simulink model "supervisor"  (R2026a)
settings: configuration reference "MCConfiguration" (kept outside this file)
settings Model: DataDictionary=embeddedBoard_common.sldd  SimulationMode=accelerator  Creator=mfussi  LastModifiedBy=rpumpo
settings ConfigSetRef: SourceName=MCConfiguration

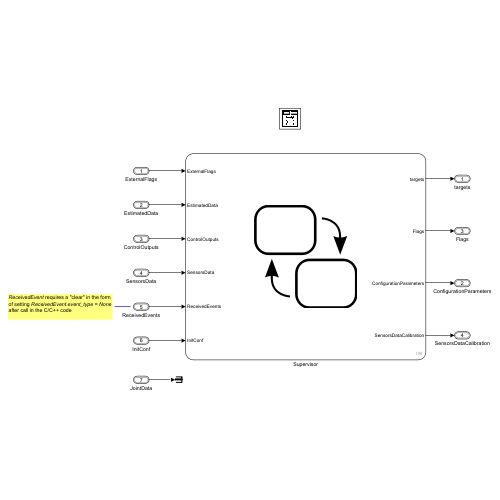
[thumbnail: Simulink's stored preview of the top-level diagram]
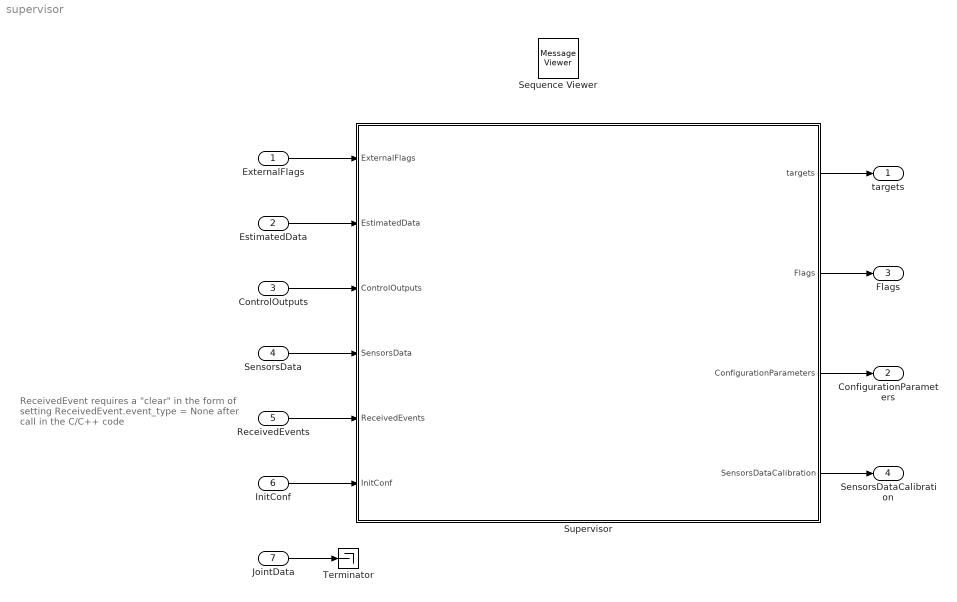
== system supervisor ==
  note: ReceivedEvent requires a "clear" in the form of setting ReceivedEvent.event_type = None after call in the C/C++ code
  ExternalFlags : Inport  OutDataTypeStr=Bus: ExternalFlags  BusOutputAsStruct=on
  EstimatedData : Inport  Port=2  OutDataTypeStr=Bus: EstimatedData  BusOutputAsStruct=on
  ControlOutputs : Inport  Port=3  OutDataTypeStr=Bus: FOCOutputs  BusOutputAsStruct=on
  SensorsData : Inport  Port=4  OutDataTypeStr=Bus: SensorsData  BusOutputAsStruct=on
  ReceivedEvents : Inport  Description=|  Port=5  OutDataTypeStr=Bus: ReceivedEvents  BusOutputAsStruct=on
      | ReceivedEvent requires a "clear" 
      | in the form of setting ReceivedEvent.event_type = None after call in the C/C++ code
  InitConf : Inport  Port=6  OutDataTypeStr=Bus: ActuatorConfiguration  BusOutputAsStruct=on
  JointData : Inport  Port=7  OutDataTypeStr=Bus: JointData
  Sequence Viewer : MessageViewer  History=1000  SavedRootId=#
  Supervisor : Stateflow chart  TreatAsAtomicUnit=on
      settings: PortSchema="{\"entries\":[{\"content\":{\"sides\":[{\"content\":{\"connectorIds\":[\"In2\",\"In1\",\"In3\",\"In4\",\"In6\",\"In5\"]},\"type\":\"ConnectorPlacement.EquallySpacedRectSide\",\"uuid\":\"924267b7-0662-4a36-add4-8ce875a6673d\"},{\"content\":{\"connectorIds\":[\"Out1\",\"Out2\",\"Out3\",\"Out4\"],\"side\":\"RIGHT\"},\"type\":\"ConnectorPlacement.EquallySpacedRectSide\",\"uuid\":\"edfdb85b-b8c0-45b0-9100-5f30a86fff38\"},{\"content\":{\"side\":\"TOP\"},\"type\":\"ConnectorPlacement.EquallySpacedRectSide\",\"uuid\":\"ff8cc695-ae52-41b0-91e9-1dc41b5aad3d\"},{\"content\":{\"side\":\"BOTTOM\"},\"type\":\"ConnectorPlacement.EquallySpacedRectSide\",\"uuid\":\"f5fe8171-8dce-40c2-ade3-2941f2e0d5a7\"}]},\"type\":\"ConnectorPlacement.EquallySpacedConnector\",\"uuid\":\"ae0a1b0b-beda-484a-966c-3dd739fb9179\"}],\"packageUris\":[\"http://schema.mathworks.com/mf0/Connector/R2020b\"],\"version\":\"1.0\"}"
  Terminator : Terminator
  targets : Outport  OutDataTypeStr=Bus: Targets  BusOutputAsStruct=on
  ConfigurationParameters : Outport  Port=2  OutDataTypeStr=Bus: ActuatorConfiguration  BusOutputAsStruct=on
  Flags : Outport  Port=3  OutDataTypeStr=Bus: Flags  BusOutputAsStruct=on
  SensorsDataCalibration : Outport  Port=4  OutDataTypeStr=Bus: SensorsData  BusOutputAsStruct=on
  wires:
  ExternalFlags/1 -> Supervisor/2(ExternalFlags)
  EstimatedData/1 -> Supervisor/1(EstimatedData)
  ControlOutputs/1 -> Supervisor/3(ControlOutputs)
  SensorsData/1 -> Supervisor/4(SensorsData)
  ReceivedEvents/1 -> Supervisor/6(ReceivedEvents)
  Supervisor/1(targets) -> targets/1
  Supervisor/3(ConfigurationParameters) -> ConfigurationParameters/1
  Supervisor/2(Flags) -> Flags/1
  InitConf/1 -> Supervisor/5(InitConf)
  JointData/1 -> Terminator/1
  Supervisor/4(SensorsDataCalibration) -> SensorsDataCalibration/1

== stateflow chart supervisor/Supervisor ==
  settings: updateMethod=DISCRETE  sampleTime=Ts_Supervision
  state FaultsManager [parallel]
    settings: executionOrder=1
    state FaultButton [parallel]
      settings: executionOrder=2
      state NoFault
        entry:
        isFaultButtonPressed = false;
      state ButtonPressed
        entry:
        isFaultButtonPressed = true;
      (default) -> FaultsManager.FaultButton.NoFault
      ButtonPressed -> FaultsManager.FaultButton.NoFault : [hasChangedTo(ExternalFlags.fault_button, false)]
      FaultsManager.FaultButton.NoFault -> ButtonPressed : [hasChangedTo(ExternalFlags.fault_button, true)]
    state HWFaults [parallel]
      settings: executionOrder=1
      state NoFault
        entry:
        isInFault=false;
        Flags.hw_faults.overcurrent = false;
      state LimitNonConfigured
      state OverCurrentFault
        entry:
        Flags.hw_faults.overcurrent = true;
        isInFault=true;
      (default) -> LimitNonConfigured
      LimitNonConfigured -> FaultsManager.HWFaults.NoFault : [areLimitsSet==true]
      FaultsManager.HWFaults.NoFault -> OverCurrentFault : [abs(EstimatedData.Iq_filtered) >= ConfigurationParameters.thresholds.motorOverloadCurrents]
      OverCurrentFault -> FaultsManager.HWFaults.NoFault : [abs(EstimatedData.Iq_filtered) < ConfigurationParameters.thresholds.motorOverloadCurrents]
  state ControlModeHandler [parallel]
    settings: executionOrder=2
    state Calibration
      entry:
      Flags.control_mode = ControlModes.Current;
      during :
      SensorsDataCalibration.motorsensors.Iabc = SensorsData.motorsensors.Iabc;
      state p_idx_out =CheckIdx(idx,p_idx) [function]
        (default) -> (junction 1789) : {diff_index = idx - p_idx;}
        (junction 1789) -> (junction 1791) [order 1] : [diff_index ~= 0]{p_idx_out = idx;}
        (junction 1789) -> (junction 1791) [order 2]
      state computed_offset = ComputeOffset(angle) [function]
        (default) -> (junction 1799) : {computed_offset = 45 - angle;}
        (junction 1799) -> (junction 1800) [order 1] : [computed_offset >360]{computed_offset = computed_offset -360;}
        (junction 1799) -> (junction 1800) [order 2]
      state Zero_electric
        entry:
        finish = false;
        p_index = SensorsData.motorsensors.qencoder.Idx_counter;
        diff_index = 0;
        tzeroalign = 0.7;
        talign = 0.01;
        v_threshold = 1;
        count = 0;
        SensorsDataCalibration.motorsensors.electrical_angle = count;
      state Search_idx
        entry:
        count = count+1;
        SensorsDataCalibration.motorsensors.electrical_angle = count;
        p_index = CheckIdx(SensorsData.motorsensors.qencoder.Idx_counter,p_index);
      state velocity_check
        newSetpoint = ConfigurationParameters.thresholds.motorNominalCurrents;
        send(ControlModeSetpointChange, TargetsManager);
      state Idx_found
        entry:
        SensorsDataCalibration.motorsensors.electrical_angle = 0;
      state Finish
        newSetpoint = 0;
        send(ControlModeSetpointChange, TargetsManager);
      state Read_0_encoder
        entry:
        offset = ComputeOffset(SensorsData.motorsensors.qencoder.rotor_angle);
      (default) -> Zero_electric : {SensorsDataCalibration = SensorsData;}
      Zero_electric -> velocity_check : [Flags.calibration_type ~= CalibrationTypes.None]{condition=1;}
      Search_idx -> Zero_electric [order 1] : [count == 360]
      velocity_check -> Search_idx [order 3] : [after(tzeroalign,sec)&& condition ==1]
      Search_idx -> velocity_check [order 3] : {condition=2;}
      velocity_check -> Search_idx [order 4] : [after(talign,sec)&&condition ==2]
      velocity_check -> velocity_check [order 2] : [abs(EstimatedData.rotor_velocity) >v_threshold]
      Search_idx -> Finish [order 2] : [diff_index~=0 && Flags.calibration_type== CalibrationTypes.Search_Index]
      velocity_check -> velocity_check [order 1] : [diff_index~=0 && Flags.calibration_type== CalibrationTypes.Full_Calibration && condition ==2]{condition= 3;}
      velocity_check -> Idx_found [order 5] : [after(talign,sec) && condition ==3]
      Idx_found -> velocity_check : {condition = 4;}
      Finish -> (junction 1818) : [after(0.1,sec)]{finish = true;}
      Read_0_encoder -> Finish
      velocity_check -> Read_0_encoder [order 6] : [after(tzeroalign,sec) && condition ==4]
    state NotConfigured
      entry:
      Flags.control_mode = ControlModes.NotConfigured;
      Flags.emit_offset_calibration = false;
      rtw_disableMotor();
    state Idle
      entry:
      Flags.control_mode = ControlModes.Idle;
      rtw_disableMotor();
      //this updates the targets value
      send(ControlModeSetpointChange, TargetsManager);
    state Position
      entry:
      Flags.control_mode = ControlModes.Position;
      newSetpoint = SensorsData.motorsensors.qencoder.rotor_angle;
      trajectoryVelocity = single(1);
      send(ControlModeSetpointChange, TargetsManager);
    state Current
      entry:
      Flags.control_mode = ControlModes.Current;
      send(ControlModeSetpointChange, TargetsManager);
    state HWFault
      entry:
      Flags.control_mode = ControlModes.HwFaultCM;
      rtw_disableMotor();
      //this updates the targets value
      send(ControlModeSetpointChange, TargetsManager);
    note: IMPORTANT:
        | Currently we use IDLE command to exit from HWFault state,
        | but We should use FORCE_IDLE command when it will be implemented
    state Voltage
      entry:
      Flags.control_mode = ControlModes.Voltage;
      send(ControlModeSetpointChange, TargetsManager);
    state Velocity
      entry:
      Flags.control_mode = ControlModes.Velocity;
      send(ControlModeSetpointChange, TargetsManager);
    (default) -> NotConfigured : {ConfigurationParameters = InitConf;}
    Calibration -> (junction 233) [order 2] : [finish]{Flags.calibration_type = CalibrationTypes.None; Flags.calibration_done = true;}
    Idle -> Calibration [order 1] : EnableCalibration
    Calibration -> (junction 233) [order 1] : [finish && Flags.calibration_type == CalibrationTypes.Full_Calibration]{Flags.calibration_type = CalibrationTypes.None; Flags.calibration_done = true;
        | ConfigurationParameters.motor.externals.rotor_index_offset = offset;
        |  Flags.emit_offset_calibration = true;}
    NotConfigured -> (junction 229) [order 1] : initialControlModeTrigger
        | {requestedControlMode = ControlModes.Idle;}
    (junction 229) -> (junction 233)
    (junction 227) -> (junction 233)
    (junction 273) -> (junction 229)
    (junction 233) -> Idle
    (junction 282) -> (junction 227)
    HWFault -> NotConfigured [order 1] : [!isInFault &&  ...
        | isReqMode(ControlModes.Idle) && ...
        | !isConfigurationSet()]
    NotConfigured -> HWFault [order 2] : [isInFault]
    (junction 228) -> Idle
    (junction 236) -> (junction 228)
    Idle -> (junction 230) [order 3] : [!isReqMode(ControlModes.Idle)]
        | {rtw_enableMotor();}
    (junction 230) -> (junction 237)
    (junction 234) -> Idle : SetCtrlMode[isReqMode(ControlModes.Idle)]
    (junction 235) -> (junction 234) [order 2]
    (junction 224) -> Idle : SetCtrlMode[isReqMode(ControlModes.Idle)]
    (junction 243) -> (junction 224) [order 2]
    (junction 231) -> Idle : SetCtrlMode[isReqMode(ControlModes.Idle)]
    (junction 241) -> (junction 231) [order 2]
    Idle -> (junction 232) [order 2] : [isInFault || isFaultButtonPressed]
    (junction 232) -> (junction 225)
    (junction 225) -> (junction 248)
    Position -> (junction 236) [order 3] : SetCtrlMode[isReqMode(ControlModes.Idle)]
    (junction 237) -> Position [order 1] : SetCtrlMode[isReqMode(ControlModes.Position)]
    (junction 237) -> (junction 244) [order 2]
    (junction 235) -> Position [order 1] : SetCtrlMode[isReqMode(ControlModes.Position)]
    (junction 245) -> (junction 235)
    Position -> (junction 242) [order 2] : SetCtrlMode[!isReqMode(ControlModes.Idle)]
    (junction 242) -> (junction 240)
    (junction 243) -> Position [order 1] : SetCtrlMode[isReqMode(ControlModes.Position)]
    (junction 247) -> (junction 243) [order 2]
    (junction 241) -> Position [order 1] : SetCtrlMode[isReqMode(ControlModes.Position)]
    (junction 255) -> (junction 241) [order 2]
    Position -> (junction 238) [order 1] : [isInFault || isFaultButtonPressed]
    (junction 238) -> (junction 248)
    (junction 248) -> (junction 259)
    (junction 244) -> Current [order 1] : SetCtrlMode[isReqMode(ControlModes.Current)]{ newSetpoint=0; }
    (junction 244) -> (junction 278) [order 2]
    Current -> (junction 245) [order 3]
    (junction 240) -> (junction 239) [order 1] : SetCtrlMode[isReqMode(ControlModes.Current)]
    (junction 239) -> Current : {newSetpoint=EstimatedData.Iq_filtered;}
    (junction 240) -> (junction 258) [order 2]
    (junction 247) -> (junction 246) [order 1] : SetCtrlMode[isReqMode(ControlModes.Current)]
    (junction 246) -> (junction 276)
    (junction 263) -> (junction 247)
    Current -> (junction 275) [order 2] : SetCtrlMode[!isReqMode(ControlModes.Idle) && !isReqMode(ControlModes.Position)]
    (junction 275) -> (junction 257)
    (junction 276) -> Current : {newSetpoint=EstimatedData.Iq_filtered;}
    (junction 255) -> (junction 276) [order 1] : SetCtrlMode[isReqMode(ControlModes.Current)]
    (junction 261) -> (junction 255) [order 2]
    HWFault -> (junction 273) [order 2] : SetCtrlMode[!isInFault && isReqMode(ControlModes.Idle)]
    Current -> (junction 267) [order 1] : [isInFault || isFaultButtonPressed]
    (junction 268) -> HWFault
    (junction 267) -> (junction 259)
    (junction 259) -> (junction 279)
    (junction 278) -> Voltage [order 1] : SetCtrlMode[isReqMode(ControlModes.Voltage)]
        | {newSetpoint=0; }
    (junction 278) -> (junction 251) [order 2]
    (junction 258) -> (junction 277) [order 1] : SetCtrlMode[isReqMode(ControlModes.Voltage)]
    (junction 277) -> Voltage : {newSetpoint=ControlOutputs.Vq;}
    (junction 258) -> (junction 251) [order 2]
    (junction 283) -> (junction 277)
    Voltage -> (junction 263) [order 2]
    (junction 257) -> (junction 283) [order 1] : SetCtrlMode[isReqMode(ControlModes.Voltage)]
    (junction 257) -> (junction 251) [order 2]
    Voltage -> (junction 251) [order 3]
    (junction 269) -> Voltage : {newSetpoint=ControlOutputs.Vq;}
    (junction 261) -> (junction 269) [order 1] : SetCtrlMode[isReqMode(ControlModes.Voltage)]
    (junction 265) -> (junction 261) : SetCtrlMode[!isReqMode(ControlModes.Velocity)]
    Voltage -> (junction 260) [order 1] : [isInFault || isFaultButtonPressed]
    (junction 260) -> (junction 279)
    (junction 279) -> (junction 253)
    (junction 251) -> Velocity : SetCtrlMode[isReqMode(ControlModes.Velocity)]
        | {newSetpoint=EstimatedData.rotor_velocity;}
    Velocity -> (junction 265) [order 2]
    Velocity -> (junction 280) [order 1] : [isInFault || isFaultButtonPressed]
    (junction 280) -> (junction 253)
    (junction 253) -> (junction 281)
    (junction 281) -> (junction 268) [order 1] : [isInFault]
    (junction 281) -> (junction 282) [order 2] : [isFaultButtonPressed]
  state TargetsManager [parallel]
    settings: executionOrder=4
    state ResetTargets [function]
      (default) -> (junction 1055) : {targets.voltage = 0;
          | targets.current = 0;
          | targets.velocity = 0;
          | targets.position = 0;
          | targets.trajectory_time = 0; }
    state Home
    (default) -> TargetsManager.Home : {ResetTargets();}
    (junction 968) -> TargetsManager.Home [order 1] : [in(ControlModeHandler.Current)| in(ControlModeHandler.Calibration)]
        | {targets.current = newSetpoint;}
    (junction 968) -> TargetsManager.Home [order 5] : [in(ControlModeHandler.Position)]
        | {targets.position = newSetpoint;
        | targets.velocity = trajectoryVelocity;}
    (junction 968) -> TargetsManager.Home [order 2] : [in(ControlModeHandler.Voltage)]
        | {targets.voltage = newSetpoint;}
    (junction 968) -> TargetsManager.Home [order 4] : [in(ControlModeHandler.Velocity)]
        | {targets.velocity = newSetpoint;}
    TargetsManager.Home -> (junction 968) [order 2] : DispatcherSetpointChange
    TargetsManager.Home -> (junction 968) [order 1] : ControlModeSetpointChange
    (junction 968) -> TargetsManager.Home [order 3] : [in(ControlModeHandler.Idle) || ...
        | in(ControlModeHandler.HWFault)]
        | {ResetTargets();}
    (junction 968) -> TargetsManager.Home [order 6] : //Default Transition
  state ConfigurationManager [parallel]
    settings: executionOrder=5
    state Home
      entry:
      param_is_set = false;
      cfg_is_set = false;
    state SetExternalConfig
      entry:
      cfg_is_set = true;
    state SetConfigParam
      entry:
      param_is_set = true;
    state wait_required = SetMotorParam(cfg_set) [function]
      (default) -> (junction 1841)
      (junction 1841) -> (junction 1842) [order 1] : [cfg_set.key == MCMotorParamsSet.Kbemf]
      (junction 1841) -> (junction 1845) [order 2]
      (junction 1842) -> (junction 1843) : {ConfigurationParameters.motor.Kbemf = cfg_set.value[0][0];
          | wait_required  = false;}
      (junction 1843) -> (junction 1844)
      (junction 1844) -> (junction 1848)
      (junction 1845) -> (junction 1846) [order 1] : [cfg_set.key == MCMotorParamsSet.elect_vmax]
      (junction 1845) -> (junction 1849) [order 2]
      (junction 1846) -> (junction 1847) : {ConfigurationParameters.motor.Vmax = cfg_set.value[0][0];
          | wait_required  = false;}
      (junction 1847) -> (junction 1848)
      (junction 1848) -> (junction 1853)
      (junction 1849) -> (junction 1850) [order 1] : [cfg_set.key == MCMotorParamsSet.hall]
      (junction 1849) -> (junction 1854) [order 2]
      (junction 1850) -> (junction 1852) : {ConfigurationParameters.motor.hall_sensors_offset = cfg_set.value[0][0];
          | ConfigurationParameters.motor.hall_sensors_swapBC = cfg_set.value[1][0];
          | wait_required  = true;}
      (junction 1852) -> (junction 1853)
      (junction 1854) -> (junction 1851)
      (junction 1853) -> (junction 1855)
      (junction 1855) -> (junction 1854)
    state CheckCalibration(motor_config) [function]
      (junction 1879) -> (junction 1878) : {offset = motor_config.rotor_index_offset;
          | has_index = motor_config.has_quadrature_encoder;}
      (default) -> (junction 1879)
      (junction 1878) -> (junction 1880)
      (junction 1880) -> (junction 1883) [order 2] : {Flags.calibration_done = true;}
      (junction 1880) -> (junction 1881) [order 1] : [has_index]{Flags.calibration_done = false;}
      (junction 1881) -> (junction 1882) [order 1] : [offset == -1]
          | {Flags.calibration_type= CalibrationTypes.Full_Calibration;}
      (junction 1881) -> (junction 1882) [order 2] : {Flags.calibration_type = CalibrationTypes.Search_Index;}
      (junction 1882) -> (junction 1883) : {send(EnableCalibration,ControlModeHandler);}
    (default) -> ConfigurationManager.Home
    ConfigurationManager.Home -> ConfigurationManager.Home [order 3] : SetMotorParam
        | [!SetMotorParam(temp_config_set)]
    ConfigurationManager.Home -> SetExternalConfig [order 1] : SetMotorConfigExternal
        | {ConfigurationParameters.motor.externals = temp_motor_config;}
    SetExternalConfig -> ConfigurationManager.Home [order 5] : [cfg_is_set]
        | {hardwareConfigMotor(motor_id_to_configure);
        | CheckCalibration(temp_motor_config);}
    SetExternalConfig -> ConfigurationManager.Home [order 1] : [hasChanged(motor_id_to_configure)]
    ConfigurationManager.Home -> SetConfigParam [order 2] : SetMotorParam
        | [SetMotorParam(temp_config_set)]
    SetConfigParam -> ConfigurationManager.Home [order 3] : [cfg_is_set]
        | {hardwareConfigMotor(motor_id_to_configure);
        | CheckCalibration(temp_motor_config);}
    SetConfigParam -> ConfigurationManager.Home [order 1] : [hasChanged(motor_id_to_configure)]
    SetExternalConfig -> SetExternalConfig [order 3] : SetMotorConfigExternal
        | {ConfigurationParameters.motor.externals = temp_motor_config;}
    SetExternalConfig -> SetExternalConfig [order 4] : SetMotorParam[!SetMotorParam(temp_config_set)]
    SetConfigParam -> SetExternalConfig [order 2] : SetMotorConfigExternal
        | {ConfigurationParameters.motor.externals = temp_motor_config;}
    SetExternalConfig -> SetConfigParam [order 2] : SetMotorParam[SetMotorParam(temp_config_set)]
    SetConfigParam -> SetConfigParam [order 4] : SetMotorParam
        | {SetMotorParam(temp_config_set);}
  state InputsDispatcher [parallel]
    settings: executionOrder=3
    state SetPid(pid) [function]
      (default) -> (junction 1523)
      (junction 1523) -> (junction 1522) [order 5]
      (junction 1523) -> (junction 1527) [order 4] : [pid.type == ControlModes.Velocity]
      (junction 1523) -> (junction 1526) [order 3] : [pid.type == ControlModes.Voltage]
      (junction 1523) -> (junction 1524) [order 1] : [pid.type == ControlModes.Current]
      (junction 1522) -> (junction 1528)
      (junction 1523) -> (junction 1525) [order 2] : [pid.type == ControlModes.Position]
      (junction 1526) -> (junction 1531) : {DirectPID.P = pid.P;
          | DirectPID.I = pid.I;
          | DirectPID.D = pid.D;
          | DirectPID.shift_factor = pid.shift_factor;}
      (junction 1527) -> (junction 1529) : {ConfigurationParameters.pids.velocityPID.P = pid.P;
          | ConfigurationParameters.pids.velocityPID.I = pid.I;
          | ConfigurationParameters.pids.velocityPID.D = pid.D;
          | ConfigurationParameters.pids.velocityPID.shift_factor = pid.shift_factor;}
      (junction 1524) -> (junction 1530) : {ConfigurationParameters.pids.currentPID.P = pid.P;
          | ConfigurationParameters.pids.currentPID.I = pid.I;
          | ConfigurationParameters.pids.currentPID.D = pid.D;
          | ConfigurationParameters.pids.currentPID.shift_factor = pid.shift_factor;
          | ConfigurationParameters.pids.currentPID.type = ControlModes.Current;}
      (junction 1525) -> (junction 1532) : {ConfigurationParameters.pids.positionPID.P = pid.P;
          | ConfigurationParameters.pids.positionPID.I = pid.I;
          | ConfigurationParameters.pids.positionPID.D = pid.D;
          | ConfigurationParameters.pids.positionPID.shift_factor = pid.shift_factor;
          | ConfigurationParameters.pids.positionPID.type = ControlModes.Position;}
      (junction 1528) -> (junction 1529)
      (junction 1529) -> (junction 1531)
      (junction 1531) -> (junction 1532)
      (junction 1530) -> (junction 1532)
    state SetTarget(tg) [function]
      (junction 1501) -> (junction 1499) [order 1] : [in(ControlModeHandler.Voltage)]{newSetpoint = tg.voltage;}
      (junction 1499) -> (junction 1500)
      (junction 1501) -> (junction 1500) [order 2] : [in(ControlModeHandler.Current)]{newSetpoint = tg.current;}
      (junction 1500) -> (junction 1502)
      (junction 1501) -> (junction 1502) [order 3] : [in(ControlModeHandler.Velocity)]{newSetpoint = tg.velocity;}
      (default) -> (junction 1501)
      (junction 1501) -> (junction 1805) [order 4] : [in(ControlModeHandler.Position)]
          | {newSetpoint = tg.position; trajectoryVelocity = tg.velocity;}
      (junction 1501) -> (junction 1503) [order 5] : [!in(ControlModeHandler.Calibration)]{newSetpoint = 0;}
      (junction 1502) -> (junction 1805)
      (junction 1805) -> (junction 1503)
      (junction 1503) -> (junction 1504) : {send(DispatcherSetpointChange, TargetsManager);}
    state SetLimits(limits) [function]
      (default) -> (junction 1516) : {ConfigurationParameters.thresholds.motorNominalCurrents = abs(limits.nominal);
          | ConfigurationParameters.thresholds.motorPeakCurrents = abs(limits.peak);
          | ConfigurationParameters.thresholds.motorOverloadCurrents = abs(limits.overload);}
      (junction 1516) -> (junction 1517) : [areLimitsSet == false]
          | {areLimitsSet = true;
          | send(initialControlModeTrigger, ControlModeHandler);}
    state Home
    (default) -> (junction 1161) : /* Consume N events per tick */
    InputsDispatcher.Home -> (junction 1161) : {Flags.enable_sending_msg_status = false;}
    (junction 1161) -> (junction 1165) : {ei = 0;}
    (junction 1165) -> (junction 1432) [order 1] : [ei < MAX_EVENTS_PER_TICK]
    (junction 1432) -> (junction 1433) [order 1] : [ReceivedEvents[ei].event_type == EventTypes.SetLimit]
        | {SetLimits(ReceivedEvents[ei].limits_content);}
    (junction 1414) -> (junction 1165) : {ei++;}
    (junction 1165) -> InputsDispatcher.Home [order 2]
    (junction 1432) -> (junction 1434) [order 2]
    (junction 1433) -> (junction 1435)
    (junction 1434) -> (junction 1435) [order 1] : [ReceivedEvents[ei].event_type == EventTypes.SetPid]
        | {SetPid(ReceivedEvents[ei].pid_content);}
    (junction 1434) -> (junction 1436) [order 2]
    (junction 1435) -> (junction 1437)
    (junction 1436) -> (junction 1437) [order 1] : [ReceivedEvents[ei].event_type == EventTypes.SetMotorConfig]
        | {temp_motor_config = ReceivedEvents[ei].motor_config_content;
        | motor_id_to_configure = ReceivedEvents[ei].motor_id;
        | send(SetMotorConfigExternal, ConfigurationManager);}
    (junction 1436) -> (junction 1438) [order 2]
    (junction 1437) -> (junction 1420)
    (junction 1438) -> (junction 1420) [order 1] : [ReceivedEvents[ei].event_type == EventTypes.SetTarget]
        | {Flags.enable_sending_msg_status = true;
        | SetTarget(ReceivedEvents[ei].targets_content);}
    (junction 1438) -> (junction 1439) [order 2]
    (junction 1420) -> (junction 1431)
    (junction 1439) -> (junction 1431) [order 1] : [ReceivedEvents[ei].event_type == EventTypes.SetControlMode]
        | {requestedControlMode = ReceivedEvents[ei].control_mode_content;
        | send(SetCtrlMode, ControlModeHandler);}
    (junction 1439) -> (junction 1904) [order 2]
    (junction 1431) -> (junction 1903)
    (junction 1904) -> (junction 1903) [order 1] : [ReceivedEvents[ei].event_type == EventTypes.SetMotorParam]
        | {temp_config_set = ReceivedEvents[ei].motor_config_set;
        | motor_id_to_configure = ReceivedEvents[ei].motor_id;
        | send(SetMotorParam, ConfigurationManager);}
    (junction 1904) -> (junction 1417) [order 2]
    (junction 1903) -> (junction 1416)
    (junction 1417) -> (junction 1416) [order 1] : [ReceivedEvents[ei].event_type == EventTypes.None]
        | { /*Skip event */ ;}
    (junction 1416) -> (junction 1414)
    (junction 1417) -> (junction 1414) [order 2]
  data: idx function_input single; p_idx function_input single; p_idx_out function_output single; angle function_input single; computed_offset function_output single; isSet function_output boolean; mode function_input Enum: ControlModes; out function_output boolean; cfg_set function_input Bus: MotorConfigurationExtSet size=1; wait_required function_output boolean; motor_id function_input uint8; motor_config function_input Bus: MotorConfigurationExternal; pid function_input Bus: PID; tg function_input Bus: Targets; limits function_input Bus: SupervisorInputLimits; ei local int32 =0; areLimitsSet local boolean; EstimatedData input Bus: EstimatedData; ExternalFlags input Bus: ExternalFlags; ControlOutputs input Bus: FOCOutputs; targets output Bus: Targets; SensorsData input Bus: SensorsData; isFaultButtonPressed local double; isInFault local double; requestedControlMode local Enum: ControlModes; newSetpoint local double; DirectPID local Bus: PID; Flags output Bus: Flags; InitConf input Bus: ActuatorConfiguration; ReceivedEvents input Bus: ReceivedEvents size=MAX_EVENTS_PER_TICK; MAX_EVENTS_PER_TICK parameter size=1; ConfigurationParameters output Bus: ActuatorConfiguration; offset local double; has_index local double; SensorsDataCalibration output Bus: SensorsData; condition local double; count local double; diff_index local single; finish local double; p_index local double; talign local double; tzeroalign local double; v_threshold local double; trajectoryVelocity local double; param_is_set local boolean; cfg_is_set local boolean; temp_motor_config local Bus: MotorConfigurationExternal; temp_config_set local Bus: MotorConfigurationExtSet; motor_id_to_configure local uint8
  events: initialControlModeTrigger local FUNCTION_CALL_EVENT; ControlModeSetpointChange local FUNCTION_CALL_EVENT; SetCtrlMode local FUNCTION_CALL_EVENT; DispatcherSetpointChange local FUNCTION_CALL_EVENT; EnableCalibration local FUNCTION_CALL_EVENT; SetMotorConfigExternal local FUNCTION_CALL_EVENT; SetMotorParam local FUNCTION_CALL_EVENT
  function isSet = isConfigurationSet:
    | function isSet = isConfigurationSet
    | 
    | % TODO: Add more conditions as more CAN packets are processed.
    | isSet = areLimitsSet; % && IsVoltageLimitSet && IsTemperatureLimitSet;
    | %isSet = isSet && a;
    | end
  function out=isReqMode(mode):
    | function out=isReqMode(mode)
    |    
    | out = (requestedControlMode == mode);
  function hardwareConfigMotor(motor_id):
    | function hardwareConfigMotor(motor_id)
    |     swapBC = uint8(ConfigurationParameters.motor.hall_sensors_swapBC);
    |     hall_sens_offset = uint16(ConfigurationParameters.motor.hall_sensors_offset * 65536/360);
    |     rtw_configMotor(motor_id, ...
    |                     cast(ConfigurationParameters.motor.externals.has_quadrature_encoder, 'uint8'),...
    |                     ConfigurationParameters.motor.externals.rotor_encoder_resolution, ...
    |                     ConfigurationParameters.motor.externals.pole_pairs, ...
    |                     cast(ConfigurationParameters.motor.externals.has_hall_sens,'uint8'), ...
    |                     swapBC, hall_sens_offset);
    | end
